simulink model "sm_cvt_power_split_pg"  (R2025a)
settings: Solver=daessc  StartTime=0.0  StopTime=25  MaxStep=0.01  RelTol=1e-3  AbsTol=1e-4  EnableMultiTasking=on
PreLoadFcn:
  | cvtPar = sm_cvt_power_split_pg_4range_param('InputOutput',HMPST);
values from neighbouring files (symbols this model uses):
  HMPST = varargin{2}    [sm_cvt_power_split_pg_4range_param.m]
undefined symbols (not defined in the file or in its folder): Local, X, Y, Z
libraries: sm_lib x7, nesl_utility x4, Multibody_Parts_Lib x3, fl_lib x2, planetary_gear_lib x1, simulink x1
CloseFcn:
  | try,close(h1_sm_planetary_gear_testrig),end
  | clear h1_sm_planetary_gear_testrig
  | 
  | clear simlog_sm_planetary_gear_testrig
  | clear logsout_sm_planetary_gear_testrig
Description:
  | Power Split Planetary Gear
  | 
  | Copyright 2023-2025 The MathWorks, Inc.
settings Model: Creator=smiller  LastModifiedBy=smiller
settings SolverCC: AutoScaleAbsTol=off  AlgebraicLoopSolver=TrustRegion
settings DataIOCC: MaxDataPoints=20000  SaveFormat=Array  ReturnWorkspaceOutputs=off  SignalLoggingName=logsout_sm_cvt_power_split_pg
settings OptimizationCC: ReuseModelBlockBuffer=off  LifeSpan=inf
settings DebuggingCC: UnderspecifiedInitializationDetection=Classic  MergeDetectMultiDrivingBlocksExec=none  SolverPrmCheckMsg=warning  UnconnectedInputMsg=warning  UnconnectedOutputMsg=warning  UnconnectedLineMsg=warning  StateNameClashWarn=warning  PregeneratedLibrarySubsystemCodeDiagnostic=none  SFUnexpectedBacktrackingDiag=warning  SFNoUnconditionalDefaultTransitionDiag=warning  SFExecutionAtInitializationDiag=none  ArithmeticOperatorsInVariantConditions=warning
settings HardwareCC: ProdBitPerPointer=32.0  ProdBitPerSizeT=32.0  ProdBitPerPtrDiffT=32.0  ProdLargestAtomicFloat=None  ProdIntDivRoundTo=Undefined  ProdEndianess=Unspecified  ProdWordSize=32.0  ProdHWDeviceType=32-bit Generic
settings ModelReferenceCC: EnableRefExpFcnMdlSchedulingChecks=on  PropagateSignalLabelsOutOfModel=off
settings SFSimCC: SimUseLocalCustomCode=off  CustomCodeUndefinedFunction=UseInterfaceOnly
settings RTWCC: RTWUseLocalCustomCode=off  GPUComputeCapability=3.5  DLArmComputeVersion=19.05
settings CodeAppCC: StateflowObjectComments=on
settings GRTTargetCC: TargetLangStandard=C89/C90 (ANSI)
settings ConfigComp: CovMetricSettings=dw  CovSaveCumulativeToWorkspaceVar=on  CovSaveSingleToWorkspaceVar=on  CovExternalEMLEnable=off
settings SimscapeCC: SimscapeNormalizeSystem=off  SimscapeLogType=all  SimscapeLogSimulationStatistics=on  SimscapeLogName=simlog_sm_cvt_power_split_pg  SimscapeLogLimitData=off  SimscapeLogDataHistory=20000.0
settings ConfigurationSet: Description=SimMechanics 2G
settings DiagnosticsConfigSet: SimMechanicsUnconnectedFramePorts=none
settings ExplorerConfigSet: InternalSimMechanicsExplorerSettings="<ExplorerConfiguration><canonicalview>default</canonicalview><AnimationSetting><BasePlaybackSpeed>1.0</BasePlaybackSpeed><PlaybackSpeedFactor>0.5</PlaybackSpeedFactor></AnimationSetting><TilePanel><TileInfo><Tiles Columns=\"1\" Count=\"1\" Rows=\"1\"><Column Weight=\"1\"/><Row Weight=\"1\"/><Tile Height=\"1\" Width=\"1\" X=\"0\" Y=\"0\"/></Tiles></TileInfo><SceneInfo><SceneViewer><BGColor><R>1</R><G>1</G><B>1</B></BGColor><Camera><DoPerspective>off</DoPerspective><Position><X>0.357710709110418301</X><Y>0.820203863271649292</Y><Z>0.422797068674006515</Z></Position><Center><X>0.00200920695206529849</X><Y>0.012066802565158203</Y><Z>-0.0466610577600518328</Z></Center><Up><X>0.920247649054262928</X><Y>-0.390538760610257829</Y><Z>-0.0249748047260850425</Z></Up><ViewLimDist>1</ViewLimDist><YLim>0.238425205654426625</YLim><XLim>0.504546268531337216</XLim></Camera></SceneViewer></SceneInfo></TilePanel><MechEditorPanel><Cameras/><GfxPanelCameraMap/><VideoCreator><PlaybackSpeedRatio>1.0</PlaybackSpeedRatio><FrameRate>30</FrameRate><VideoFormat>MPEG-4</VideoFormat><FrameSize>auto</FrameSize></VideoCreator></MechEditorPanel></ExplorerConfiguration>"

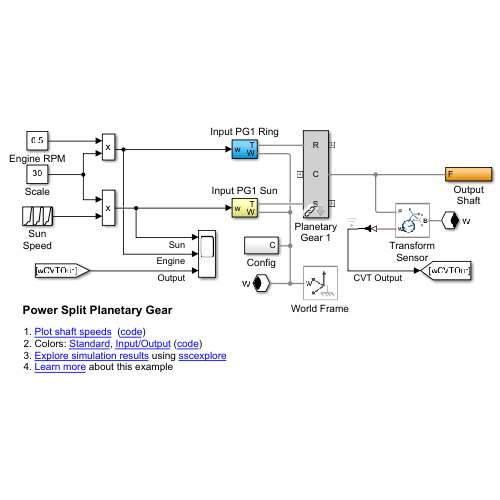
[thumbnail: Simulink's stored preview of the top-level diagram]
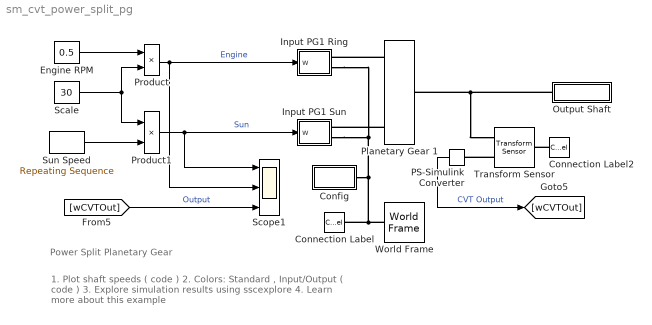
== system sm_cvt_power_split_pg ==
  note: Power Split Planetary Gear
  note: 1. Plot shaft speeds ( code )
      | 2. Colors: Standard , Input/Output ( code )
      | 3. Explore simulation results using sscexplore
      | 4. Learn more about this example
  Config : Subsystem
  Connection Label : ConnectionLabel  Label=W
  Connection Label2 : ConnectionLabel  Label=W
  Engine RPM : Constant  Value=0.5
  Input PG1 Ring : Subsystem  Tag=PublishSubsystem
  Input PG1 Sun : Subsystem  Tag=PublishSubsystem
  Output Shaft : Subsystem
  PS-Simulink Converter : nesl_utility/PS-Simulink Converter  PhysicalDomain=network_engine_domain  SubClassName=ps_output  LeftPortType=input  RightPortType=output  PseudoPeriodic=off  Frequencies=[]  VectorFormat=inherit  Unit=rpm  AffineConversion=off
  Planetary Gear 1 : planetary_gear_lib/Planetary Gear  Tag=PublishSubsystem  rad_sun=cvtPar.pg1_sun_rad  nteeth_sun=cvtPar.pg1_sun_nteeth  rad_planet=cvtPar.pg1_pla_rad  nteeth_planet=cvtPar.pg1_pla_nteeth  rad_ring=2*cvtPar.pg1_pla_rad+cvtPar.pg1_sun_rad  nteeth_ring=cvtPar.pg1_rin_nteeth  pg_axial_offset=cvtPar.plaGear_axial_offset  gear_thickness=cvtPar.gear_thickness  link_thickness=cvtPar.link_thickness  rad_hole=cvtPar.rad_hole  ring_gear_clr=cvtPar.clr.pg1.ring  sun_gear_clr=cvtPar.clr.pg1.sun  pla_gear_clr=cvtPar.clr.pg1.pla  carrier_color=cvtPar.clr.pg4.carr
  Product : Product
  Product1 : Product
  Scale : Constant  Value=30
  Scope1 : Scope  NumInputPorts=3
      settings: ActiveDisplayYMinimum=-75  ActiveDisplayYMaximum=75
  Sun Speed : simulink/Sources/Repeating Sequence  rep_seq_t=[0 5 10 15 20 25]  rep_seq_y=[-2 -2 -1.2685 -1.2685 2 2]
  Transform Sensor : sm_lib/Frames and Transforms/Transform Sensor  MeasurementFrame=World  RotationSequence=XYX  SenseAngle=off  SenseAxis=off  SenseQ=off  SenseR=off  SenseRotationSequence=off  SenseOmegaX=off  SenseOmegaY=off  SenseOmegaZ=on  SenseOmega=off  SenseQDot=off  SenseRDot=off  SenseRotationSequenceDot=off  SenseAlphaX=off  SenseAlphaY=off  SenseAlphaZ=off  SenseAlpha=off  SenseQDDot=off  SenseRDDot=off  SenseX=off  SenseY=off  SenseZ=off  SenseXYZ=off  SenseRad=off  SenseAzim=off  SenseDist=off  SenseInc=off  SenseXDot=off  SenseYDot=off  SenseZDot=off  SenseXYZDot=off  SenseRadDot=off  SenseAzimDot=off  SenseDistDot=off  SenseIncDot=off  SenseXDDot=off  SenseYDDot=off  SenseZDDot=off  SenseXYZDDot=off  SenseRadDDot=off  SenseAzimDDot=off  SenseDistDDot=off  SenseIncDDot=off
  World Frame : sm_lib/Frames and Transforms/World Frame
  wires:
  PS-Simulink Converter/1 -> [wCVTOut]  "CVT Output"
  Engine RPM/1 -> Product/1
  Sun Speed/1 -> Product1/2
  Scale/1 -> Product1/1, Product/2
  Product/1 -> Input PG1 Ring/1(w), Scope1/2  "Engine"
  Product1/1 -> Input PG1 Sun/1(w), Scope1/1  "Sun"
  [wCVTOut] -> Scope1/3  "Output"
  connections:
  Planetary Gear 1/LConn3 -- Input PG1 Sun/RConn1
  Planetary Gear 1/LConn1 -- Input PG1 Ring/RConn1
  World Frame/RConn1 -- Connection Label/LConn1 -- Config/LConn1 -- Input PG1 Sun/RConn2 -- Input PG1 Ring/RConn2
  Output Shaft/RConn1 -- Transform Sensor/RConn1 -- Planetary Gear 1/RConn2
  Connection Label2/LConn1 -- Transform Sensor/LConn1
  Transform Sensor/RConn2 -- PS-Simulink Converter/LConn1

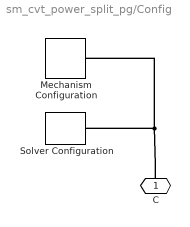
== system sm_cvt_power_split_pg/Config ==
  Mechanism Configuration : sm_lib/Utilities/Mechanism Configuration  UniformGravity=Constant  GravityVector=[0 0 0]  GravityVectorUnits=m/s^2  LinearizationDelta=0.001  JointModeTransitionNonlinearIterations=2
  Solver Configuration : nesl_utility/Solver Configuration  PhysicalDomain=network_engine_domain  SubClassName=solver  LeftPortType=input  RightPortType=generic  Tones=[]  Harmonics=[]  SimulateNoise=off  Profile=off  UseLocalSampling=off  EnableSwitchedLinearOptims=on  FrequencyDomain=off  UseCCode=off  RelTol=0.001  AbsTol=1e-06  MinStep=1e-09  ToWorkspace=off  RevertToSquareIcSolve=off  NumHomotopyIterations=100  PhasorMode=off  PhasorModeNumHarmonics=1  ConsistencySolver=NEWTON_FTOL  IndexReductionMethod=DerivativeReplacement  DoDC=off  ResidualTolerance=1e-9  ConsistencyTolSource=GLOBAL  ConsistencyAbsTol=0.001  ConsistencyRelTol=0.001  ConsistencyTolFactor=0.001  UseLocalSolver=off  LocalSolverChoice=NE_BACKWARD_EULER_ADVANCER  ResolveIndetEquations=on  FunctionEvalNumThread=1  LocalSolverSampleTime=.001  DoFixedCost=off  MaxNonlinIter=3  MaxModeIter=2  ComputeImpulses=off  ImpulseIterations=2  LinearAlgebra=Sparse  LinearAlgebraNumThread=0  EquationFormulation=NE_TIME_EF  DelaysMemoryBudget=1024  AutomaticFiltering=on  FilteringTimeConstant=0.001  PartitionStorageMethod=AS_NEEDED  PartitionMemoryBudget=1024  PartitionMethod=FAST  MultibodyUseLocalSolver=off  MultibodyLocalSolverChoice=ODE1  MultibodyLocalSolverSampleTime=0.001
  C : PMIOPort  Side=Left
  connections:
  Mechanism Configuration/RConn1 -- Solver Configuration/RConn1 -- C/RConn1

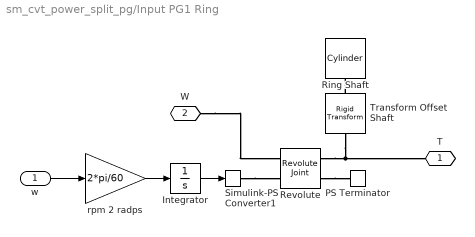
== system sm_cvt_power_split_pg/Input PG1 Ring ==
  w : Inport
  Integrator : Integrator
  PS Terminator : fl_lib/Physical Signals/Sinks/PS Terminator
  Revolute : sm_lib/Joints/Revolute Joint  JointMode=Normal  CompositeWrenchDir=FollowerOnBase  CompositeWrenchFrame=BaseFrame  SenseConstraintForce=off  SenseConstraintTorque=off  SenseTotalForce=off  SenseTotalTorque=off  PositionTargetSpecify=off  PositionTargetPriority=High  PositionTargetValue=0  PositionTargetValueUnits=deg  VelocityTargetSpecify=off  VelocityTargetPriority=High  VelocityTargetValue=0  VelocityTargetValueUnits=deg/s  EquilibriumPosition=0  EquilibriumPositionUnits=deg  SpringStiffness=0  SpringStiffnessUnits=N*m/deg  DampingCoefficient=0  DampingCoefficientUnits=N*m/(deg/s)  LowerLimitSpecify=off  LowerLimitBound=-90  LowerLimitBoundUnits=deg  LowerLimitStiffness=1e4  LowerLimitStiffnessUnits=N*m/deg  LowerLimitDamping=10  LowerLimitDampingUnits=N*m/(deg/s)  LowerLimitTransitionRegionWidth=0.1  LowerLimitTransitionRegionWidthUnits=deg  UpperLimitSpecify=off  UpperLimitBound=90  UpperLimitBoundUnits=deg  UpperLimitStiffness=1e4  UpperLimitStiffnessUnits=N*m/deg  UpperLimitDamping=10  UpperLimitDampingUnits=N*m/(deg/s)  UpperLimitTransitionRegionWidth=0.1  UpperLimitTransitionRegionWidthUnits=deg  TorqueActuationMode=ComputedTorque  MotionActuationMode=InputMotion  SensePosition=off  SenseVelocity=on  SenseAcceleration=off  SenseTorqueForce=off  SenseLowerLimitTorqueForce=off  SenseUpperLimitTorqueForce=off
  Ring Shaft : Multibody_Parts_Lib/Basic/Cylinder  cyl_ra=cvtPar.rad_hole*6  cyl_th=cvtPar.gear_thickness*1  cyl_hr=cvtPar.rad_hole*3  cyl_rho=7000  cyl_clr=cvtPar.clr.pg1.ring  cyl_opc=1  popup_markings=Two  mark_radius_range=[0.7 0.9]  mark_angle_range=60  mark_color=[1 1 1]
  Simulink-PS Converter1 : nesl_utility/Simulink-PS Converter  PhysicalDomain=network_engine_domain  SubClassName=ps_input  LeftPortType=input  RightPortType=output  PseudoPeriodic=off  Frequencies=[]  NoiseDistribution=none  NoiseParameters=[]  Unit=rad  AffineConversion=off  FilteringAndDerivatives=filter  SimscapeFilterOrder=2  InputFilterTimeConstant=0.001  UdotUserProvided=0
  Transform Offset Shaft : sm_lib/Frames and Transforms/Rigid Transform  RotationMethod=None  FollAlignAxisA=+X  BaseAlignAxisA=+Y  FollAlignAxisB=+Y  BaseAlignAxisB=+Z  RotationStandardAxis=+Z  RotationAngle=0.0  RotationAngleUnits=deg  RotationArbitraryAxis=[0 0 1]  RotationSequenceAxes=FollowerAxes  RotationSequence=XYX  RotationSequenceAngles=[0 0 0]  RotationSequenceAnglesUnits=deg  RotationMatrix=[1 0 0; 0 1 0; 0 0 1]  Quaternion=[1 0 0 0]  TranslationMethod=StandardAxis  TranslationCartesianOffset=[0 0 0]  TranslationCartesianOffsetUnits=m  TranslationStandardAxis=+Z  TranslationStandardOffset=cvtPar.gear_thickness*3  TranslationStandardOffsetUnits=m  TranslationROffset=0  TranslationROffsetUnits=m  TranslationThetaOffset=0  TranslationThetaOffsetUnits=deg  TranslationZOffset=0  TranslationZOffsetUnits=m
  rpm 2 radps : Gain  Gain=2*pi/60
  T : PMIOPort  Side=Right
  W : PMIOPort  Port=2  Side=Right
  wires:
  Integrator/1 -> Simulink-PS Converter1/1
  w/1 -> rpm 2 radps/1
  rpm 2 radps/1 -> Integrator/1
  connections:
  Simulink-PS Converter1/RConn1 -- Revolute/LConn2
  Revolute/RConn2 -- PS Terminator/LConn1
  Revolute/RConn1 -- T/RConn1 -- Transform Offset Shaft/RConn1
  W/RConn1 -- Revolute/LConn1
  Transform Offset Shaft/LConn1 -- Ring Shaft/RConn1

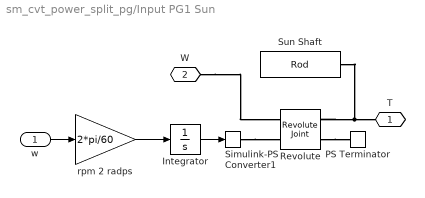
== system sm_cvt_power_split_pg/Input PG1 Sun ==
  w : Inport
  Integrator : Integrator
  PS Terminator : fl_lib/Physical Signals/Sinks/PS Terminator
  Revolute : sm_lib/Joints/Revolute Joint  JointMode=Normal  CompositeWrenchDir=FollowerOnBase  CompositeWrenchFrame=BaseFrame  SenseConstraintForce=off  SenseConstraintTorque=off  SenseTotalForce=off  SenseTotalTorque=off  PositionTargetSpecify=off  PositionTargetPriority=High  PositionTargetValue=0  PositionTargetValueUnits=deg  VelocityTargetSpecify=off  VelocityTargetPriority=High  VelocityTargetValue=0  VelocityTargetValueUnits=deg/s  EquilibriumPosition=0  EquilibriumPositionUnits=deg  SpringStiffness=0  SpringStiffnessUnits=N*m/deg  DampingCoefficient=0  DampingCoefficientUnits=N*m/(deg/s)  LowerLimitSpecify=off  LowerLimitBound=-90  LowerLimitBoundUnits=deg  LowerLimitStiffness=1e4  LowerLimitStiffnessUnits=N*m/deg  LowerLimitDamping=10  LowerLimitDampingUnits=N*m/(deg/s)  LowerLimitTransitionRegionWidth=0.1  LowerLimitTransitionRegionWidthUnits=deg  UpperLimitSpecify=off  UpperLimitBound=90  UpperLimitBoundUnits=deg  UpperLimitStiffness=1e4  UpperLimitStiffnessUnits=N*m/deg  UpperLimitDamping=10  UpperLimitDampingUnits=N*m/(deg/s)  UpperLimitTransitionRegionWidth=0.1  UpperLimitTransitionRegionWidthUnits=deg  TorqueActuationMode=ComputedTorque  MotionActuationMode=InputMotion  SensePosition=off  SenseVelocity=on  SenseAcceleration=off  SenseTorqueForce=off  SenseLowerLimitTorqueForce=off  SenseUpperLimitTorqueForce=off
  Simulink-PS Converter1 : nesl_utility/Simulink-PS Converter  PhysicalDomain=network_engine_domain  SubClassName=ps_input  LeftPortType=input  RightPortType=output  PseudoPeriodic=off  Frequencies=[]  NoiseDistribution=none  NoiseParameters=[]  Unit=rad  AffineConversion=off  FilteringAndDerivatives=filter  SimscapeFilterOrder=2  InputFilterTimeConstant=0.001  UdotUserProvided=0
  Sun Shaft : Multibody_Parts_Lib/Basic/Rod  rod_rad=cvtPar.rad_hole*2  rod_len=cvtPar.gear_thickness*5  rod_rho=7000  rod_color=cvtPar.clr.pg1.sun  rod_opc=1  popup_zori=Local +Z  popup_markings=None  mark_radius_range=[0.5 1.01]  mark_length_range=1.005  mark_angle_range=30  mark_color=[1 1 1]
  rpm 2 radps : Gain  Gain=2*pi/60
  T : PMIOPort  Side=Right
  W : PMIOPort  Port=2  Side=Right
  wires:
  w/1 -> rpm 2 radps/1
  Integrator/1 -> Simulink-PS Converter1/1
  rpm 2 radps/1 -> Integrator/1
  connections:
  W/RConn1 -- Revolute/LConn1
  Revolute/RConn1 -- Sun Shaft/RConn1 -- T/RConn1
  Revolute/RConn2 -- PS Terminator/LConn1
  Simulink-PS Converter1/RConn1 -- Revolute/LConn2

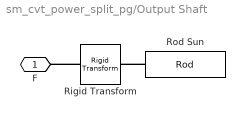
== system sm_cvt_power_split_pg/Output Shaft ==
  Rigid Transform : sm_lib/Frames and Transforms/Rigid Transform  RotationMethod=None  FollAlignAxisA=+X  BaseAlignAxisA=+Y  FollAlignAxisB=+Y  BaseAlignAxisB=+Z  RotationStandardAxis=+Z  RotationAngle=0.0  RotationAngleUnits=deg  RotationArbitraryAxis=[0 0 1]  RotationSequenceAxes=FollowerAxes  RotationSequence=XYX  RotationSequenceAngles=[0 0 0]  RotationSequenceAnglesUnits=deg  RotationMatrix=[1 0 0; 0 1 0; 0 0 1]  Quaternion=[1 0 0 0]  TranslationMethod=StandardAxis  TranslationCartesianOffset=[0 0 0]  TranslationCartesianOffsetUnits=m  TranslationStandardAxis=+Z  TranslationStandardOffset=-cvtPar.plaGear_axial_offset+cvtPar.gear_thickness  TranslationStandardOffsetUnits=m  TranslationROffset=0  TranslationROffsetUnits=m  TranslationThetaOffset=0  TranslationThetaOffsetUnits=deg  TranslationZOffset=0  TranslationZOffsetUnits=m
  Rod Sun : Multibody_Parts_Lib/Basic/Rod  rod_rad=cvtPar.rad_hole*2  rod_len=cvtPar.gear_thickness  rod_rho=7000  rod_color=cvtPar.clr.pg4.carr  rod_opc=1  popup_zori=Local +Z  popup_markings=None  mark_radius_range=[0.5 1.01]  mark_length_range=1.005  mark_angle_range=30  mark_color=[1 1 1]
  F : PMIOPort  Side=Right
  connections:
  Rigid Transform/LConn1 -- F/RConn1
  Rod Sun/LConn1 -- Rigid Transform/RConn1
